simulink model "ackermann02"  (R2026a)
settings: Solver=VariableStepAuto  StopTime=20.0
undefined symbols (not defined in the file): radarD, radarX
libraries: robotmobilelib x1, simulink x1
settings Model: Creator=hanjiatong  LastModifiedBy=hanjiatong

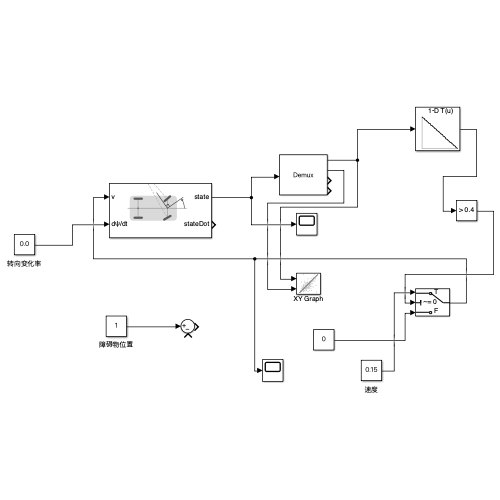
[thumbnail: Simulink's stored preview of the top-level diagram]
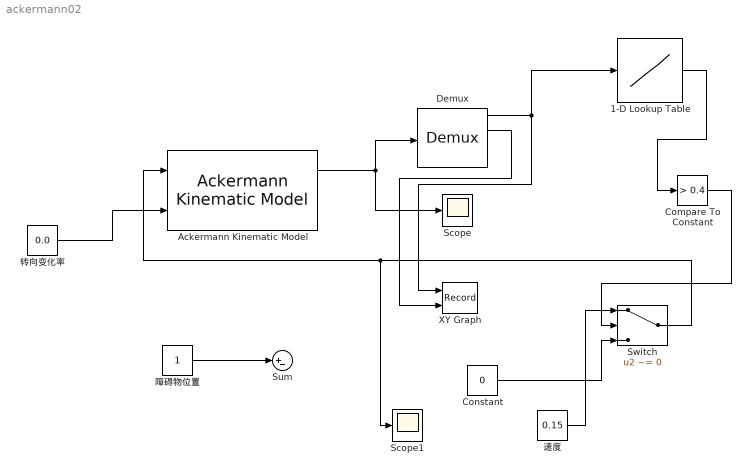
== system ackermann02 ==
  1-D Lookup Table : Lookup_n-D  NumberOfTableDimensions=1  BreakpointsForDimension1=radarX  Table=radarD  ExtrapMethod=Clip  InternalRulePriority=Speed  RndMeth=Simplest
  Ackermann Kinematic Model : robotmobilelib/Ackermann Kinematic Model  WheelBase=0.144  VehicleSpeedRange=[-inf inf]  MaxSteeringAngle=pi/4  InitialState=[0.5; 1.5; 0; 0]  SimulateUsing=Interpreted execution
  Compare To Constant : simulink/Logic and Bit Operations/Compare To Constant  relop=>  const=0.4  OutDataTypeStr=boolean
  Constant : Constant  Value=0
  Demux : Demux
      settings: DisplayOption=none
  Scope : Scope
      settings: ActiveDisplayYMinimum=-0.19594221664657985  ActiveDisplayYMaximum=1.7514452129987257
  Scope1 : Scope
  Sum : Sum  Inputs=|+-
  Switch : Switch  Criteria=u2 ~= 0  SaturateOnIntegerOverflow=off  InputSameDT=off
  XY Graph : Record  NumPorts=2.0  FileSettingsInternal="{\"entries\":[{\"content\":{\"excelSettings\":{\"content\":{},\"type\":\"Streamout.ExcelSettings\"},\"parquetSettings\":{\"content\":{},\"type\":\"Streamout.ParquetSettings\"}},\"type\":\"Streamout.FileSettingStorage\",\"uuid\":\"\"}],\"packageUris\":[\"http:\\/\\/schema.mathworks.com\\/mf0\\/streamout_blocks\\/R2020a\"],\"version\":\"1.0\"}"  FrameSettings=[0, 0]  Layout=[1 1]  SignalsInternal="{\"entries\":[{\"content\":{\"signals\":[{\"content\":{\"blockPath\":[],\"dimensions\":[1],\"domain\":\"\",\"lineColor\":\"#a2142f\",\"plots\":[ 1 ],\"port\":1,\"sid\":[\"\"],\"signalID\":1,\"signalName\":\"Demux:1\"},\"type\":\"RecordBlkView.Signal\",\"uuid\":\"\"},{\"content\":{\"blockPath\":[],\"dimensions\":[1],\"domain\":\"\",\"lineColor\":\"#139fff\",\"plots\":[ 1 ],\"port\":2,\"sid\":[\"\"],\"signalID\":2,\"signalName\":\"Demux:2\"},\"type\":\"RecordBlkView.Signal\",\"uuid\":\"\"}]},\"type\":\"RecordBlkView.InputSignals\",\"uuid\":\"\"}],\"packageUris\":[\"http:\\/\\/schema.mathworks.com\\/mf0\\/streamout_blocks\\/R2020a\"],\"version\":\"1.0\"}"  VisualizationBindings="{\"xyplotplugin\":{\"info\":[{\"series\":[{\"bindingParametersList\":[{\"parameter\":\"X-Axis\",\"signalID\":1,\"signalName\":\"Demux:1\"},{\"parameter\":\"Y-Axis\",\"signalID\":2,\"signalName\":\"Demux:2\"}],\"seriesID\":0}],\"subplotID\":1}]}}"  CompatibilityTag=XY
  转向变化率 : Constant  Value=0.0
  速度 : Constant  Value=0.15
  障碍物位置 : Constant
  wires:
  转向变化率/1 -> Ackermann Kinematic Model/2
  Ackermann Kinematic Model/1 -> Scope/1, Demux/1
  Demux/1 -> XY Graph/1, 1-D Lookup Table/1
  Demux/2 -> XY Graph/2
  障碍物位置/1 -> Sum/1
  Switch/1 -> Scope1/1, Ackermann Kinematic Model/1
  Compare To Constant/1 -> Switch/2
  速度/1 -> Switch/1
  Constant/1 -> Switch/3
  1-D Lookup Table/1 -> Compare To Constant/1
